simulink model "pmpc_mil_nu"  (R2024b)
settings: Solver=ode1  StartTime=0  StopTime=20  FixedStep=0.001  RelTol=1e-3
PreLoadFcn:
  | root = 'D:\OneDrive - mail.scut.edu.cn\Thesis\Code\Controller\MAIN\experiments\nonuniform_grid_20261115';
  | 
  | addpath(fullfile(root,'pmpc_core'),'-begin');
  | addpath(fullfile(root,'nlcsnn'),'-begin');
values from neighbouring files (symbols this model uses):
  a_pl = exp(-Tc/tau_e)    [init_valve2.m]
  b_pl = (Vdc/R)*(1 - a_pl)    [init_valve2.m]
  Iref_init = 0    [init_valve2.m]
  Ki = wc*R/Vdc    (= 26.1799387799)    [init_valve2.m]
  Kp = Ti_ratio*wc*L_H/Vdc    (= 0.0418879020479)    [init_valve2.m]
  Tc = 1/fs_ctrl    (= 0.001)    [init_valve2.m]
  Ts_avg = Tc    (= 0.001)    [init_valve2.m]
undefined symbols (not defined in the file or in its folder): delta_d, dspblkCoreblockFVToolHelper, gcbh, params, Reftraj, state0, V_target
libraries: slpidlib x5, Solver_SF x1
settings Model: Creator=user  LastModifiedBy=user
settings OptimizationCC: ZeroExternalMemoryAtStartup=off  ZeroInternalMemoryAtStartup=off
settings RTWCC: TargetLang=C++
settings GRTTargetCC: TargetLangStandard=C++11 (ISO)  CodeInterfacePackaging=C++ class

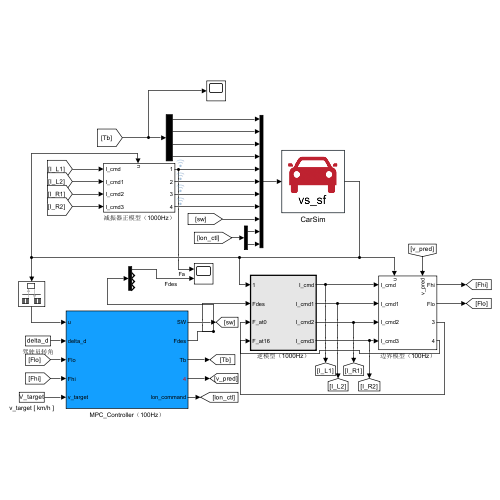
[thumbnail: Simulink's stored preview of the top-level diagram]
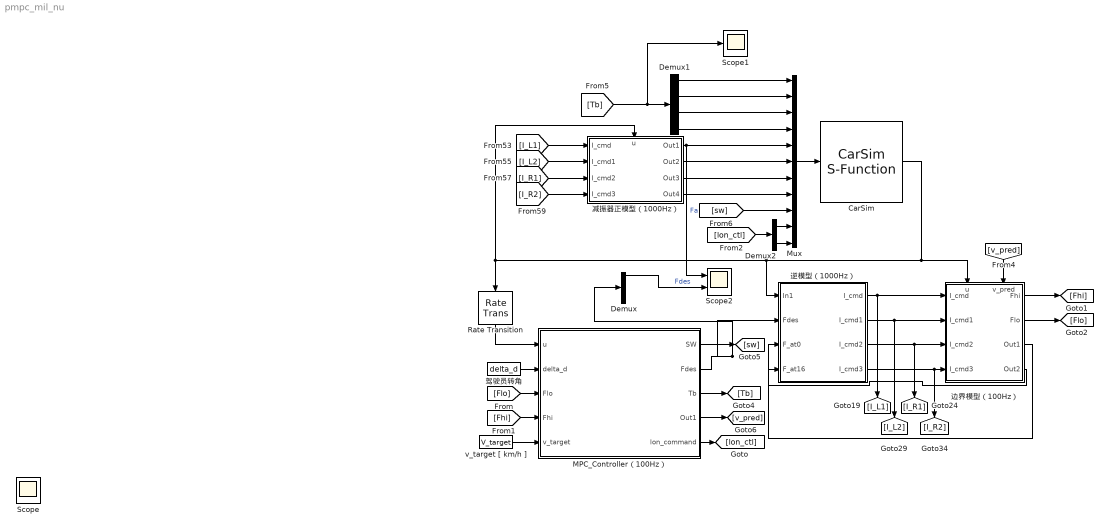
== system pmpc_mil_nu ==
  CarSim : Solver_SF/CarSim S-Function  Priority=1  SIMFILE=simfile.sim
  Demux : Demux
  Demux1 : Demux
  Demux2 : Demux  Outputs=2
  MPC_Controller（100Hz） : Subsystem  SystemSampleTime=0.01
  Mux : Mux  Inputs=11
  Rate Transition : RateTransition  OutPortSampleTime=0.01
  Scope1 : Scope
  Scope2 : Scope  NumInputPorts=2
  v_target [ km/h ] : Constant  Value=V_target
  减振器正模型（1000Hz） : Subsystem
      settings: PortSchema="{\"entries\":[{\"content\":{\"sides\":[{\"content\":{\"connectorIds\":[\"In1\",\"In2\",\"In3\",\"In4\"]},\"type\":\"ConnectorPlacement.EquallySpacedRectSide\",\"uuid\":\"6bdae15d-f673-492b-8508-25b25c52f85c\"},{\"content\":{\"connectorIds\":[\"Out1\",\"Out2\",\"Out3\",\"Out4\"],\"side\":\"RIGHT\"},\"type\":\"ConnectorPlacement.EquallySpacedRectSide\",\"uuid\":\"9d0d46be-4d90-4429-bc90-e3747ae06ca5\"},{\"content\":{\"connectorIds\":[\"In5\"],\"side\":\"TOP\"},\"type\":\"ConnectorPlacement.EquallySpacedRectSide\",\"uuid\":\"d2f3a784-c5ed-41f2-ae04-a2222bae6aeb\"}]},\"type\":\"ConnectorPlacement.EquallySpacedConnector\",\"uuid\":\"c35c18e7-51b3-4d33-8294-a9e611d66578\"}],\"packageUris\":[\"http://schema.mathworks.com/mf0/Connector/R2020b\"],\"version\":\"1.0\"}"
  边界模型（100Hz） : Subsystem
      settings: PortSchema="{\"entries\":[{\"content\":{\"sides\":[{\"content\":{\"connectorIds\":[\"In1\",\"In2\",\"In3\",\"In4\"]},\"type\":\"ConnectorPlacement.EquallySpacedRectSide\",\"uuid\":\"717c1422-5e21-4652-bca5-057ad50c6cdf\"},{\"content\":{\"connectorIds\":[\"Out1\",\"Out2\",\"Out3\",\"Out4\"],\"side\":\"RIGHT\"},\"type\":\"ConnectorPlacement.EquallySpacedRectSide\",\"uuid\":\"4ad5078c-896a-44f2-a1cc-d2c9341f0df9\"},{\"content\":{\"connectorIds\":[\"In5\",\"In6\"],\"side\":\"TOP\"},\"type\":\"ConnectorPlacement.EquallySpacedRectSide\",\"uuid\":\"81dc3538-7b06-42f0-8b15-8c4302fdfcb3\"}]},\"type\":\"ConnectorPlacement.EquallySpacedConnector\",\"uuid\":\"666a4fc5-cde4-42f5-84f2-e20b6be44764\"}],\"packageUris\":[\"http://schema.mathworks.com/mf0/Connector/R2020b\"],\"version\":\"1.0\"}"
  逆模型（1000Hz） : Subsystem  TreatAsAtomicUnit=on  SystemSampleTime=0.001
  驾驶员转角 : Constant  Value=delta_d
  Scope : Scope
  wires:
  Mux/1 -> CarSim/1
  [I_L1] -> 减振器正模型（1000Hz）/1(I_cmd)
  [I_L2] -> 减振器正模型（1000Hz）/2(I_cmd1)
  [I_R1] -> 减振器正模型（1000Hz）/3(I_cmd2)
  [I_R2] -> 减振器正模型（1000Hz）/4(I_cmd3)
  [sw] -> Mux/9
  减振器正模型（1000Hz）/1(Out1) -> Mux/5, Scope2/1  "Fa"
  减振器正模型（1000Hz）/2(Out2) -> Mux/6
  减振器正模型（1000Hz）/3(Out3) -> Mux/7
  减振器正模型（1000Hz）/4(Out4) -> Mux/8
  Demux1/1 -> Mux/1
  Demux1/2 -> Mux/2
  Demux1/3 -> Mux/3
  Demux1/4 -> Mux/4
  CarSim/1 -> 边界模型（100Hz）/5(u), 逆模型（1000Hz）/1(In1), 减振器正模型（1000Hz）/5(u), Rate Transition/1
  [Flo] -> MPC_Controller（100Hz）/3(Flo)
  [Fhi] -> MPC_Controller（100Hz）/4(Fhi)
  MPC_Controller（100Hz）/3(Tb) -> [Tb]
  MPC_Controller（100Hz）/1(SW) -> [sw]
  Rate Transition/1 -> MPC_Controller（100Hz）/1(u)
  逆模型（1000Hz）/1(I_cmd) -> [I_L1], 边界模型（100Hz）/1(I_cmd)
  逆模型（1000Hz）/2(I_cmd1) -> [I_L2], 边界模型（100Hz）/2(I_cmd1)
  逆模型（1000Hz）/3(I_cmd2) -> [I_R1], 边界模型（100Hz）/3(I_cmd2)
  逆模型（1000Hz）/4(I_cmd3) -> [I_R2], 边界模型（100Hz）/4(I_cmd3)
  MPC_Controller（100Hz）/2(Fdes) -> Demux/1, 逆模型（1000Hz）/2(Fdes)
  v_target [ km/h ]/1 -> MPC_Controller（100Hz）/5(v_target)
  [Tb] -> Scope1/1, Demux1/1
  边界模型（100Hz）/1(Fhi) -> [Fhi]
  边界模型（100Hz）/2(Flo) -> [Flo]
  MPC_Controller（100Hz）/4(Out1) -> [v_pred]
  [v_pred] -> 边界模型（100Hz）/6(v_pred)
  Demux/1 -> Scope2/2  "Fdes"
  MPC_Controller（100Hz）/5(lon_command) -> [lon_ctl]
  Demux2/1 -> Mux/10
  Demux2/2 -> Mux/11
  [lon_ctl] -> Demux2/1
  驾驶员转角/1 -> MPC_Controller（100Hz）/2(delta_d)
  边界模型（100Hz）/3(Out1) -> 逆模型（1000Hz）/3(F_at0)
  边界模型（100Hz）/4(Out2) -> 逆模型（1000Hz）/4(F_at16)

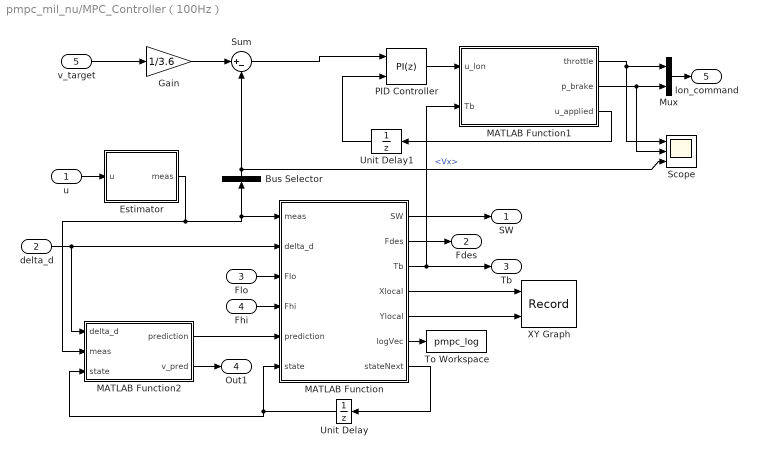
== system pmpc_mil_nu/MPC_Controller（100Hz） ==
  u : Inport
  delta_d : Inport  Port=2
  Flo : Inport  Port=3
  Fhi : Inport  Port=4
  v_target : Inport  Port=5
  Bus Selector : BusSelector  OutputSignals=Vx
  Estimator : MATLAB Function  TreatAsAtomicUnit=on
  Gain : Gain  Gain=1/3.6
  MATLAB Function : MATLAB Function  TreatAsAtomicUnit=on
  MATLAB Function1 : MATLAB Function  TreatAsAtomicUnit=on
  MATLAB Function2 : MATLAB Function  TreatAsAtomicUnit=on
  Mux : Mux  Inputs=2
  PID Controller : slpidlib/PID Controller  Controller=PI  Form=Parallel  TimeDomain=Discrete-time  UseExternalTs=off  SampleTime=-1  IntegratorMethod=Forward Euler  FilterMethod=Forward Euler  ControllerParametersSource=internal  P=0.2  I=0.005  UseKiTs=off  D=0  UseExternalDerivativeSource=off  N=100  UseFilter=on  TunerSelectOption=Transfer Function Based (PID Tuner App)  InitialConditionSource=internal  InitialConditionForIntegrator=0  InitialConditionForFilter=0  DifferentiatorICPrevScaledInput=0  ExternalReset=none  TrackingMode=on  Kt=1  LimitOutput=on  SatLimitsSource=internal  UpperSaturationLimit=1  LowerSaturationLimit=-1  LinearizeAsGain=on  AntiWindupMode=back-calculation  Kb=1  LimitIntegrator=off  UpperIntegratorSaturationLimit=inf  LowerIntegratorSaturationLimit=-inf  POutMin=[]  POutMax=[]  IOutMin=[]  IOutMax=[]  DOutMin=[]  DOutMax=[]  NOutMin=[]  NOutMax=[]  SumOutMin=[]  SumOutMax=[]  SaturationOutMin=[]  SaturationOutMax=[]  PParamMin=[]  PParamMax=[]  IParamMin=[]  IParamMax=[]  DParamMin=[]  DParamMax=[]  NParamMin=[]  NParamMax=[]  KbParamMin=[]  KbParamMax=[]  KtParamMin=[]  KtParamMax=[]  KbOutMin=[]  KbOutMax=[]  KtOutMin=[]  KtOutMax=[]  IntegratorOutMin=[]  IntegratorOutMax=[]  FilterOutMin=[]  FilterOutMax=[]  SumI1OutMin=[]  SumI1OutMax=[]  SumI2OutMin=[]  SumI2OutMax=[]  SumI3OutMin=[]  SumI3OutMax=[]  SumI4OutMin=[]  SumI4OutMax=[]  SumDOutMin=[]  SumDOutMax=[]  DifferentiatorOutMin=[]  DifferentiatorOutMax=[]  FilterDiffOutCoefMin=[]  FilterDiffOutCoefMax=[]  ReciprocalOutMin=[]  ReciprocalOutMax=[]  SumDenOutMin=[]  SumDenOutMax=[]  SumNumOutMin=[]  SumNumOutMax=[]  DivideOutMin=[]  DivideOutMax=[]  UdiffTsProdOutMin=[]  UdiffTsProdOutMax=[]  NTsProdOutMin=[]  NTsProdOutMax=[]  UintegralTsProdOutMin=[]  UintegralTsProdOutMax=[]  UngainTsProdOutMin=[]  UngainTsProdOutMax=[]  ClampingZeroOutDataTypeStr=Inherit: Inherit via back propagation  ClampingZeroOutMin=[]  ClampingZeroOutMax=[]  FilterDenConstantOutDataTypeStr=Inherit: Inherit via back propagation  FilterDenConstantOutMin=[]  FilterDenConstantOutMax=[]  PCopyOutDataTypeStr=Inherit: Inherit via back propagation  PCopyOutMin=[]  PCopyOutMax=[]  NCopyOutDataTypeStr=Inherit: Inherit via back propagation  NCopyOutMin=[]  NCopyOutMax=[]  IntegratorContinuousStateAttributes=''  IntegratorStateMustResolveToSignalObject=off  IntegratorRTWStateStorageClass=Auto  FilterContinuousStateAttributes=''  FilterStateMustResolveToSignalObject=off  FilterRTWStateStorageClass=Auto  ParallelPVariant=InternalParameters  IdealPVariant=Disabled  IVariant=InternalParameters  DVariant=Disabled  IntegratorVariant=Discrete  SatVariant=Enabled  AWVariant=BackCalculation  PCopyVariant=Disabled  TRVariant=Enabled  FdbkBlocksVariant=Forward  IdealPFdbkVariant=Disabled  SatFdbkVariant=Disabled  DerivativeFilterVariant=Disabled  NVariant=Disabled  NCopyVariant=Disabled_SignalSpec  FilterICVariant=Disabled  IntegratorICVariant=InternalICs  ExternalResetVariant=Disabled  TRSumVariant=TrackingMode  SumFdbkVariant=Disabled  SumVariant=Sum_PI  TsampFilterVariant=InternalTs  TsampNgainVariant=Passthrough  TsampIntegralVariant=Disabled_SignalSpec  ExternalSaturationOutDataTypeStr=Inherit: Same as second input  DerivativeSourceVariant=Disabled  PreIntVariant=InternalPreInt
  Scope : Scope  NumInputPorts=3
  Sum : Sum  Inputs=|+-
  To Workspace : ToWorkspace  VariableName=pmpc_log  SaveFormat=Timeseries  SampleTime=-1
  Unit Delay : UnitDelay  InitialCondition=state0  SampleTime=0.01  HasFrameUpgradeWarning=on
  Unit Delay1 : UnitDelay  SampleTime=-1  HasFrameUpgradeWarning=on
  XY Graph : Record  FileSettingsInternal="{\"entries\":[{\"content\":{\"excelSettings\":{\"content\":{},\"type\":\"Streamout.ExcelSettings\"}},\"type\":\"Streamout.FileSettingStorage\",\"uuid\":\"\"}],\"packageUris\":[\"http:\\/\\/schema.mathworks.com\\/mf0\\/streamout_blocks\\/R2020a\"],\"version\":\"1.0\"}"  Layout=[1 1]  SignalsInternal="{\"entries\":[{\"content\":{\"signals\":[{\"content\":{\"blockPath\":[],\"dimensions\":[1],\"domain\":\"\",\"lineColor\":\"#a2142f\",\"lineWidth\":2,\"plots\":[ 1 ],\"port\":1,\"signalID\":1,\"signalName\":\"MATLAB Function:4\"},\"type\":\"RecordBlkView.Signal\",\"uuid\":\"\"},{\"content\":{\"blockPath\":[],\"dimensions\":[1],\"domain\":\"\",\"lineColor\":\"#139fff\",\"lineWidth\":2,\"plots\":[ 1 ],\"port\":2,\"signalID\":2,\"signalName\":\"MATLAB Function:5\"},\"type\":\"RecordBlkView.Signal\",\"uuid\":\"\"}]},\"type\":\"RecordBlkView.InputSignals\",\"uuid\":\"\"}],\"packageUris\":[\"http:\\/\\/schema.mathworks.com\\/mf0\\/streamout_blocks\\/R2020a\"],\"version\":\"1.0\"}"  VisualizationBindings="{\"xyplotplugin\":{\"info\":[{\"series\":[{\"bindingParametersList\":[{\"parameter\":\"X-Axis\",\"signalID\":1,\"signalName\":\"MATLAB Function:4\"},{\"parameter\":\"Y-Axis\",\"signalID\":2,\"signalName\":\"MATLAB Function:5\"}],\"seriesID\":0}],\"subplotID\":1}]}}"  CompatibilityTag=XY
  SW : Outport
  Fdes : Outport  Port=2
  Tb : Outport  Port=3
  Out1 : Outport  Port=4
  lon_command : Outport  Port=5
  wires:
  u/1 -> Estimator/1(u)
  Estimator/1(meas) -> MATLAB Function2/2(meas), Bus Selector/1, MATLAB Function/1(meas)
  Unit Delay/1 -> MATLAB Function/6(state), MATLAB Function2/3(state)
  MATLAB Function/7(stateNext) -> Unit Delay/1
  Flo/1 -> MATLAB Function/3(Flo)
  Fhi/1 -> MATLAB Function/4(Fhi)
  Sum/1 -> PID Controller/1
  PID Controller/1 -> MATLAB Function1/1(u_lon)
  Bus Selector/1 -> Sum/2, Scope/3  "<Vx>"
  v_target/1 -> Gain/1
  MATLAB Function1/2(p_brake) -> Mux/2, Scope/2
  Gain/1 -> Sum/1
  MATLAB Function1/3(u_applied) -> Unit Delay1/1
  Unit Delay1/1 -> PID Controller/2
  MATLAB Function1/1(throttle) -> Mux/1, Scope/1
  MATLAB Function/1(SW) -> SW/1
  MATLAB Function/3(Tb) -> Tb/1, MATLAB Function1/2(Tb)
  MATLAB Function/2(Fdes) -> Fdes/1
  MATLAB Function/4(Xlocal) -> XY Graph/1
  MATLAB Function/5(Ylocal) -> XY Graph/2
  MATLAB Function2/1(prediction) -> MATLAB Function/5(prediction)
  MATLAB Function2/2(v_pred) -> Out1/1
  Mux/1 -> lon_command/1
  MATLAB Function/6(logVec) -> To Workspace/1
  delta_d/1 -> MATLAB Function2/1(delta_d), MATLAB Function/2(delta_d)

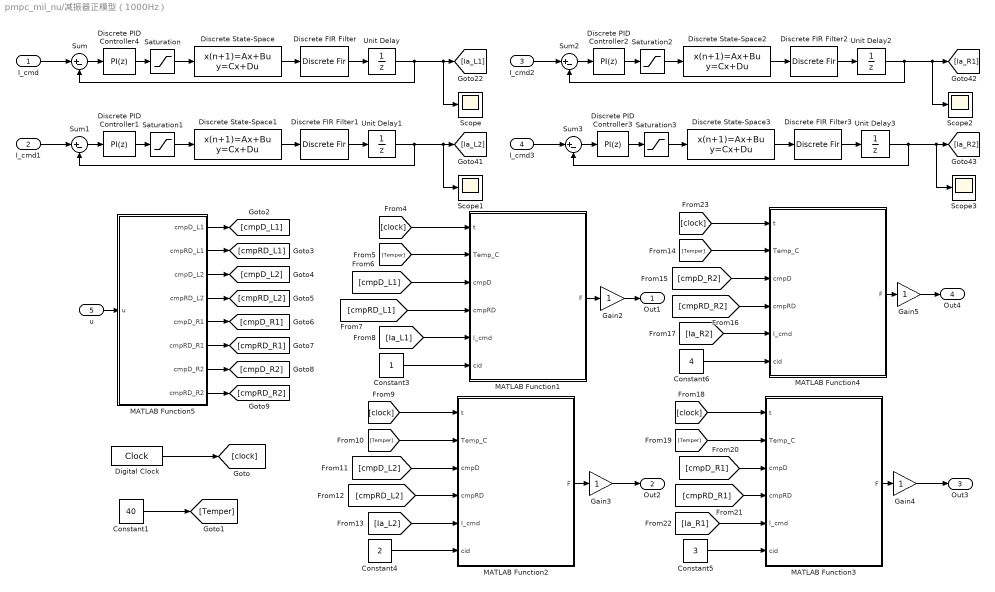
== system pmpc_mil_nu/减振器正模型（1000Hz） ==
  I_cmd : Inport
  I_cmd1 : Inport  Port=2
  I_cmd2 : Inport  Port=3
  I_cmd3 : Inport  Port=4
  u : Inport  Port=5
  Constant1 : Constant  Value=40
  Constant3 : Constant
  Constant4 : Constant  Value=2
  Constant5 : Constant  Value=3
  Constant6 : Constant  Value=4
  Digital Clock : DigitalClock  SampleTime=0.001
  Discrete FIR Filter{,1..3} (4 alike) : DiscreteFir  LoadFcn=dspblkCoreblockFVToolHelper(gcbh,'load');  InitialStates=Iref_init
      settings: CopyFcn=dspblkCoreblockFVToolHelper(gcbh,'copy');  DeleteFcn=dspblkCoreblockFVToolHelper(gcbh,'close');  ModelCloseFcn=dspblkCoreblockFVToolHelper(gcbh,'close');  PreSaveFcn=dspblkCoreblockFVToolHelper(gcbh,'presave');  PostSaveFcn=dspblkCoreblockFVToolHelper(gcbh,'postsave');  CloseFcn=dspblkCoreblockFVToolHelper(gcbh,'close');
  Discrete PID Controller{1..4} (4 alike) : slpidlib/PID Controller  Controller=PI  Form=Parallel  TimeDomain=Discrete-time  UseExternalTs=off  SampleTime=Tc  IntegratorMethod=Forward Euler  FilterMethod=Forward Euler  ControllerParametersSource=internal  P=Kp  I=Ki  UseKiTs=off  D=0  UseExternalDerivativeSource=off  N=100  UseFilter=on  TunerSelectOption=Transfer Function Based (PID Tuner App)  InitialConditionSource=internal  InitialConditionForIntegrator=D_init  InitialConditionForFilter=0  DifferentiatorICPrevScaledInput=0  ExternalReset=none  TrackingMode=off  Kt=1  LimitOutput=on  SatLimitsSource=internal  UpperSaturationLimit=1  LowerSaturationLimit=0  LinearizeAsGain=off  AntiWindupMode=clamping  Kb=1  LimitIntegrator=off  UpperIntegratorSaturationLimit=duty_max − u_ff  LowerIntegratorSaturationLimit=duty_min − u_ff  POutMin=[]  POutMax=[]  IOutMin=[]  IOutMax=[]  DOutMin=[]  DOutMax=[]  NOutMin=[]  NOutMax=[]  SumOutMin=[]  SumOutMax=[]  SaturationOutMin=[]  SaturationOutMax=[]  PParamMin=[]  PParamMax=[]  IParamMin=[]  IParamMax=[]  DParamMin=[]  DParamMax=[]  NParamMin=[]  NParamMax=[]  KbParamMin=[]  KbParamMax=[]  KtParamMin=[]  KtParamMax=[]  KbOutMin=[]  KbOutMax=[]  KtOutMin=[]  KtOutMax=[]  IntegratorOutMin=[]  IntegratorOutMax=[]  FilterOutMin=[]  FilterOutMax=[]  SumI1OutMin=[]  SumI1OutMax=[]  SumI2OutMin=[]  SumI2OutMax=[]  SumI3OutMin=[]  SumI3OutMax=[]  SumI4OutMin=[]  SumI4OutMax=[]  SumDOutMin=[]  SumDOutMax=[]  DifferentiatorOutMin=[]  DifferentiatorOutMax=[]  FilterDiffOutCoefMin=[]  FilterDiffOutCoefMax=[]  ReciprocalOutMin=[]  ReciprocalOutMax=[]  SumDenOutMin=[]  SumDenOutMax=[]  SumNumOutMin=[]  SumNumOutMax=[]  DivideOutMin=[]  DivideOutMax=[]  UdiffTsProdOutMin=[]  UdiffTsProdOutMax=[]  NTsProdOutMin=[]  NTsProdOutMax=[]  UintegralTsProdOutMin=[]  UintegralTsProdOutMax=[]  UngainTsProdOutMin=[]  UngainTsProdOutMax=[]  ClampingZeroOutDataTypeStr=Inherit: Inherit via back propagation  ClampingZeroOutMin=[]  ClampingZeroOutMax=[]  FilterDenConstantOutDataTypeStr=Inherit: Inherit via back propagation  FilterDenConstantOutMin=[]  FilterDenConstantOutMax=[]  PCopyOutDataTypeStr=Inherit: Inherit via back propagation  PCopyOutMin=[]  PCopyOutMax=[]  NCopyOutDataTypeStr=Inherit: Inherit via back propagation  NCopyOutMin=[]  NCopyOutMax=[]  IntegratorContinuousStateAttributes=''  IntegratorStateMustResolveToSignalObject=off  IntegratorRTWStateStorageClass=Auto  FilterContinuousStateAttributes=''  FilterStateMustResolveToSignalObject=off  FilterRTWStateStorageClass=Auto  ParallelPVariant=InternalParameters  IdealPVariant=Disabled  IVariant=InternalParameters  DVariant=Disabled  IntegratorVariant=Discrete  SatVariant=Enabled  AWVariant=DiscClampingParallel  PCopyVariant=Disabled  TRVariant=Disabled  FdbkBlocksVariant=Forward  IdealPFdbkVariant=Disabled  SatFdbkVariant=Disabled  DerivativeFilterVariant=Disabled  NVariant=Disabled  NCopyVariant=Disabled_SignalSpec  FilterICVariant=Disabled  IntegratorICVariant=InternalICs  ExternalResetVariant=Disabled  TRSumVariant=Passthrough  SumFdbkVariant=Disabled  SumVariant=Sum_PI  TsampFilterVariant=InternalTs  TsampNgainVariant=Passthrough  TsampIntegralVariant=Disabled_SignalSpec  ExternalSaturationOutDataTypeStr=Inherit: Same as second input  DerivativeSourceVariant=Disabled  PreIntVariant=InternalPreInt
      settings: LibrarySourceBlock=simulink/Discrete/Discrete PID Controller
  Discrete State-Space{,1..3} (4 alike) : DiscreteStateSpace  A=a_pl  B=b_pl  D=0  InitialCondition=Iref_init  SampleTime=Ts_avg
  Gain{2..5} (4 alike) : Gain
  MATLAB Function1 : MATLAB Function  TreatAsAtomicUnit=on
  MATLAB Function2 : MATLAB Function  TreatAsAtomicUnit=on
  MATLAB Function3 : MATLAB Function  TreatAsAtomicUnit=on
  MATLAB Function4 : MATLAB Function  TreatAsAtomicUnit=on
  MATLAB Function5 : MATLAB Function  TreatAsAtomicUnit=on
  Saturation{,1..3} (4 alike) : Saturate  UpperLimit=1  LowerLimit=0
  Scope{,1..3} (4 alike) : Scope
  Sum{,1..3} (4 alike) : Sum  Inputs=|+-
  Unit Delay{,1..3} (4 alike) : UnitDelay  InitialCondition=Iref_init  SampleTime=1e-3  HasFrameUpgradeWarning=on
  Out1 : Outport
  Out2 : Outport  Port=2
  Out3 : Outport  Port=3
  Out4 : Outport  Port=4
  wires:
  [clock] -> MATLAB Function4/1(t)
  [Ia_R2] -> MATLAB Function4/5(I_cmd)
  Constant5/1 -> MATLAB Function3/6(cid)
  [Temper] -> MATLAB Function1/2(Temp_C)
  MATLAB Function1/1(F) -> Gain2/1
  [cmpRD_R1] -> MATLAB Function3/4(cmpRD)
  [Ia_R1] -> MATLAB Function3/5(I_cmd)
  [Ia_L1] -> MATLAB Function1/5(I_cmd)
  [clock] -> MATLAB Function3/1(t)
  [Ia_L2] -> MATLAB Function2/5(I_cmd)
  Constant4/1 -> MATLAB Function2/6(cid)
  MATLAB Function2/1(F) -> Gain3/1
  [cmpD_R2] -> MATLAB Function4/3(cmpD)
  Digital Clock/1 -> [clock]
  Gain3/1 -> Out2/1
  [cmpRD_L1] -> MATLAB Function1/4(cmpRD)
  Gain5/1 -> Out4/1
  [Temper] -> MATLAB Function3/2(Temp_C)
  MATLAB Function3/1(F) -> Gain4/1
  Constant1/1 -> [Temper]
  [cmpRD_L2] -> MATLAB Function2/4(cmpRD)
  [cmpD_R1] -> MATLAB Function3/3(cmpD)
  [cmpRD_R2] -> MATLAB Function4/4(cmpRD)
  Gain4/1 -> Out3/1
  [clock] -> MATLAB Function1/1(t)
  MATLAB Function4/1(F) -> Gain5/1
  [cmpD_L1] -> MATLAB Function1/3(cmpD)
  Gain2/1 -> Out1/1
  Constant6/1 -> MATLAB Function4/6(cid)
  [Temper] -> MATLAB Function2/2(Temp_C)
  Constant3/1 -> MATLAB Function1/6(cid)
  [Temper] -> MATLAB Function4/2(Temp_C)
  [clock] -> MATLAB Function2/1(t)
  [cmpD_L2] -> MATLAB Function2/3(cmpD)
  u/1 -> MATLAB Function5/1(u)
  MATLAB Function5/1(cmpD_L1) -> [cmpD_L1]
  MATLAB Function5/2(cmpRD_L1) -> [cmpRD_L1]
  MATLAB Function5/3(cmpD_L2) -> [cmpD_L2]
  MATLAB Function5/4(cmpRD_L2) -> [cmpRD_L2]
  MATLAB Function5/5(cmpD_R1) -> [cmpD_R1]
  MATLAB Function5/6(cmpRD_R1) -> [cmpRD_R1]
  MATLAB Function5/7(cmpD_R2) -> [cmpD_R2]
  MATLAB Function5/8(cmpRD_R2) -> [cmpRD_R2]
  I_cmd/1 -> Sum/1
  Sum/1 -> Discrete PID Controller4/1
  Unit Delay/1 -> Scope/1, [Ia_L1], Sum/2
  Discrete FIR Filter/1 -> Unit Delay/1
  Discrete PID Controller4/1 -> Saturation/1
  Discrete State-Space/1 -> Discrete FIR Filter/1
  Saturation/1 -> Discrete State-Space/1
  Unit Delay1/1 -> [Ia_L2], Scope1/1, Sum1/2
  Discrete State-Space1/1 -> Discrete FIR Filter1/1
  Discrete FIR Filter1/1 -> Unit Delay1/1
  Saturation1/1 -> Discrete State-Space1/1
  Sum1/1 -> Discrete PID Controller1/1
  Discrete PID Controller1/1 -> Saturation1/1
  Unit Delay2/1 -> [Ia_R1], Scope2/1, Sum2/2
  Discrete State-Space2/1 -> Discrete FIR Filter2/1
  Discrete FIR Filter2/1 -> Unit Delay2/1
  Saturation2/1 -> Discrete State-Space2/1
  Sum2/1 -> Discrete PID Controller2/1
  Discrete PID Controller2/1 -> Saturation2/1
  Unit Delay3/1 -> [Ia_R2], Scope3/1, Sum3/2
  Discrete State-Space3/1 -> Discrete FIR Filter3/1
  Discrete FIR Filter3/1 -> Unit Delay3/1
  Saturation3/1 -> Discrete State-Space3/1
  Sum3/1 -> Discrete PID Controller3/1
  I_cmd3/1 -> Sum3/1
  Discrete PID Controller3/1 -> Saturation3/1
  I_cmd1/1 -> Sum1/1
  I_cmd2/1 -> Sum2/1

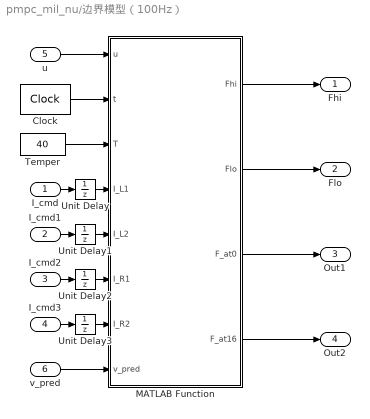
== system pmpc_mil_nu/边界模型（100Hz） ==
  I_cmd : Inport
  I_cmd1 : Inport  Port=2
  I_cmd2 : Inport  Port=3
  I_cmd3 : Inport  Port=4
  u : Inport  Port=5
  v_pred : Inport  Port=6
  Clock : DigitalClock  SampleTime=0.001
  MATLAB Function : MATLAB Function  TreatAsAtomicUnit=on
  Temper : Constant  Value=40
  Unit Delay{,1..3} (4 alike) : UnitDelay  SampleTime=0.001  HasFrameUpgradeWarning=on
  Fhi : Outport
  Flo : Outport  Port=2
  Out1 : Outport  Port=3
  Out2 : Outport  Port=4
  wires:
  Temper/1 -> MATLAB Function/3(T)
  Clock/1 -> MATLAB Function/2(t)
  v_pred/1 -> MATLAB Function/8(v_pred)
  u/1 -> MATLAB Function/1(u)
  MATLAB Function/1(Fhi) -> Fhi/1
  MATLAB Function/2(Flo) -> Flo/1
  I_cmd/1 -> Unit Delay/1
  Unit Delay/1 -> MATLAB Function/4(I_L1)
  I_cmd1/1 -> Unit Delay1/1
  Unit Delay1/1 -> MATLAB Function/5(I_L2)
  I_cmd2/1 -> Unit Delay2/1
  Unit Delay2/1 -> MATLAB Function/6(I_R1)
  I_cmd3/1 -> Unit Delay3/1
  Unit Delay3/1 -> MATLAB Function/7(I_R2)
  MATLAB Function/3(F_at0) -> Out1/1
  MATLAB Function/4(F_at16) -> Out2/1

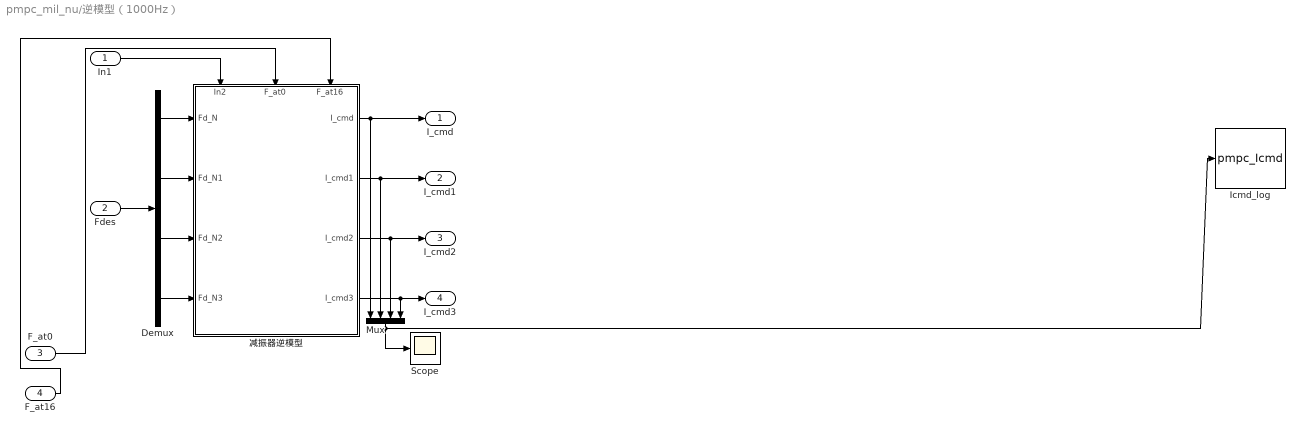
== system pmpc_mil_nu/逆模型（1000Hz） ==
  In1 : Inport
  Fdes : Inport  Port=2
  F_at0 : Inport  Port=3
  F_at16 : Inport  Port=4
  Demux : Demux
  Icmd_log : ToWorkspace  VariableName=pmpc_Icmd  SaveFormat=Structure With Time  SampleTime=-1
  Mux : Mux
  Scope : Scope
  减振器逆模型 : Subsystem
      settings: PortSchema="{\"entries\":[{\"content\":{\"sides\":[{\"content\":{\"connectorIds\":[\"In1\",\"In2\",\"In3\",\"In4\"]},\"type\":\"ConnectorPlacement.EquallySpacedRectSide\",\"uuid\":\"1b1e3cbb-ab52-4b5e-a8c1-091191c7a0a1\"},{\"content\":{\"connectorIds\":[\"Out1\",\"Out2\",\"Out3\",\"Out4\"],\"side\":\"RIGHT\"},\"type\":\"ConnectorPlacement.EquallySpacedRectSide\",\"uuid\":\"e36391e6-cb8e-45c5-b600-19fb73252ab2\"},{\"content\":{\"connectorIds\":[\"In5\",\"In6\",\"In7\"],\"side\":\"TOP\"},\"type\":\"ConnectorPlacement.EquallySpacedRectSide\",\"uuid\":\"92f6e0c3-7b8a-4a08-9013-fccb1e083f6f\"}]},\"type\":\"ConnectorPlacement.EquallySpacedConnector\",\"uuid\":\"3214107d-4344-4e68-82b7-79bb17f5024d\"}],\"packageUris\":[\"http://schema.mathworks.com/mf0/Connector/R2020b\"],\"version\":\"1.0\"}"
  I_cmd : Outport
  I_cmd1 : Outport  Port=2
  I_cmd2 : Outport  Port=3
  I_cmd3 : Outport  Port=4
  wires:
  Demux/2 -> 减振器逆模型/2(Fd_N1)
  Demux/4 -> 减振器逆模型/4(Fd_N3)
  减振器逆模型/2(I_cmd1) -> I_cmd1/1, Mux/2
  Demux/1 -> 减振器逆模型/1(Fd_N)
  Demux/3 -> 减振器逆模型/3(Fd_N2)
  In1/1 -> 减振器逆模型/5(In2)
  减振器逆模型/1(I_cmd) -> I_cmd/1, Mux/1
  减振器逆模型/4(I_cmd3) -> I_cmd3/1, Mux/4
  减振器逆模型/3(I_cmd2) -> I_cmd2/1, Mux/3
  Fdes/1 -> Demux/1
  Mux/1 -> Scope/1, Icmd_log/1
  F_at0/1 -> 减振器逆模型/6(F_at0)
  F_at16/1 -> 减振器逆模型/7(F_at16)

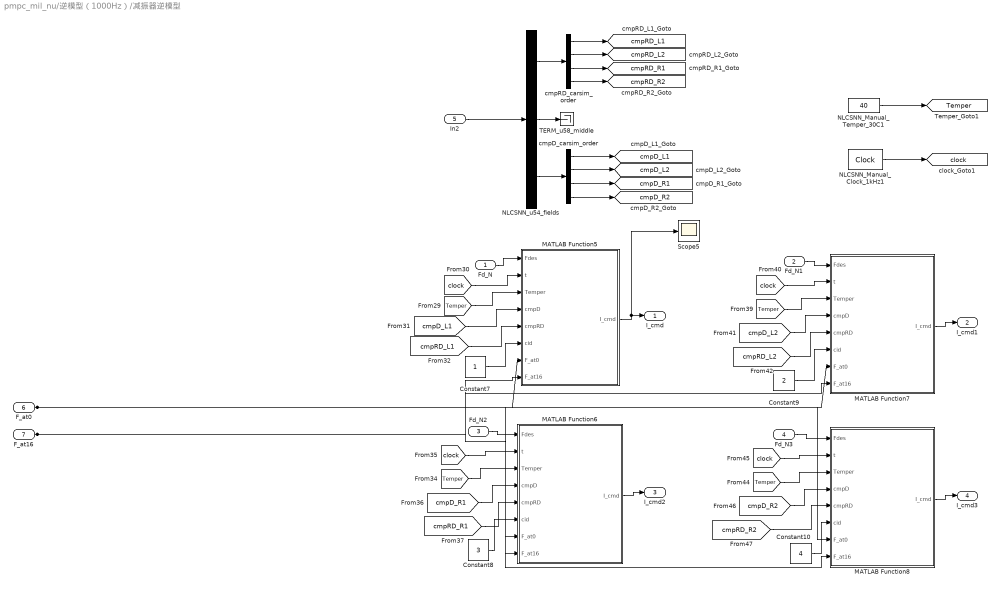
== system pmpc_mil_nu/逆模型（1000Hz）/减振器逆模型 ==
  Fd_N : Inport
  Fd_N1 : Inport  Port=2
  Fd_N2 : Inport  Port=3
  Fd_N3 : Inport  Port=4
  In2 : Inport  Port=5
  F_at0 : Inport  Port=6
  F_at16 : Inport  Port=7
  Constant10 : Constant  Value=4
  Constant7 : Constant
  Constant8 : Constant  Value=3
  Constant9 : Constant  Value=2
  MATLAB Function5 : MATLAB Function  TreatAsAtomicUnit=on
  MATLAB Function6 : MATLAB Function  TreatAsAtomicUnit=on
  MATLAB Function7 : MATLAB Function  TreatAsAtomicUnit=on
  MATLAB Function8 : MATLAB Function  TreatAsAtomicUnit=on
  NLCSNN_Manual_Clock_1kHz1 : DigitalClock  SampleTime=0.001
  NLCSNN_Manual_Temper_30C1 : Constant  Value=40
  NLCSNN_u54_fields : Demux  Outputs=[4 46 4]
  Scope5 : Scope
  TERM_u58_middle : Terminator
  cmpD_carsim_order : Demux
  cmpRD_carsim_order : Demux
  I_cmd : Outport
  I_cmd1 : Outport  Port=2
  I_cmd2 : Outport  Port=3
  I_cmd3 : Outport  Port=4
  tag scope: Temper=global, clock=global, cmpD_L1=global, cmpD_L2=global, cmpD_R1=global, cmpD_R2=global, cmpRD_L1=global, cmpRD_L2=global, cmpRD_R1=global, cmpRD_R2=global
  wires:
  [cmpD_R2] -> MATLAB Function8/4(cmpD)
  [Temper] -> MATLAB Function6/3(Temper)
  In2/1 -> NLCSNN_u54_fields/1
  Constant9/1 -> MATLAB Function7/6(cid)
  [cmpRD_R1] -> MATLAB Function6/5(cmpRD)
  [Temper] -> MATLAB Function5/3(Temper)
  [clock] -> MATLAB Function8/2(t)
  NLCSNN_u54_fields/1 -> cmpRD_carsim_order/1
  Fd_N/1 -> MATLAB Function5/1(Fdes)
  [cmpD_L1] -> MATLAB Function5/4(cmpD)
  cmpD_carsim_order/2 -> [cmpD_L2]
  NLCSNN_u54_fields/2 -> TERM_u58_middle/1
  Fd_N2/1 -> MATLAB Function6/1(Fdes)
  Constant8/1 -> MATLAB Function6/6(cid)
  [cmpRD_L1] -> MATLAB Function5/5(cmpRD)
  cmpRD_carsim_order/4 -> [cmpRD_R2]
  cmpRD_carsim_order/2 -> [cmpRD_L2]
  cmpD_carsim_order/1 -> [cmpD_L1]
  MATLAB Function7/1(I_cmd) -> I_cmd1/1
  MATLAB Function5/1(I_cmd) -> I_cmd/1, Scope5/1
  cmpRD_carsim_order/1 -> [cmpRD_L1]
  cmpD_carsim_order/3 -> [cmpD_R1]
  cmpRD_carsim_order/3 -> [cmpRD_R1]
  NLCSNN_u54_fields/3 -> cmpD_carsim_order/1
  cmpD_carsim_order/4 -> [cmpD_R2]
  [clock] -> MATLAB Function5/2(t)
  [clock] -> MATLAB Function6/2(t)
  [cmpRD_L2] -> MATLAB Function7/5(cmpRD)
  [clock] -> MATLAB Function7/2(t)
  Constant7/1 -> MATLAB Function5/6(cid)
  [cmpRD_R2] -> MATLAB Function8/5(cmpRD)
  Constant10/1 -> MATLAB Function8/6(cid)
  [Temper] -> MATLAB Function7/3(Temper)
  NLCSNN_Manual_Clock_1kHz1/1 -> [clock]
  NLCSNN_Manual_Temper_30C1/1 -> [Temper]
  [Temper] -> MATLAB Function8/3(Temper)
  [cmpD_R1] -> MATLAB Function6/4(cmpD)
  [cmpD_L2] -> MATLAB Function7/4(cmpD)
  MATLAB Function8/1(I_cmd) -> I_cmd3/1
  Fd_N1/1 -> MATLAB Function7/1(Fdes)
  Fd_N3/1 -> MATLAB Function8/1(Fdes)
  MATLAB Function6/1(I_cmd) -> I_cmd2/1
  F_at0/1 -> MATLAB Function5/7(F_at0), MATLAB Function6/7(F_at0), MATLAB Function7/7(F_at0), MATLAB Function8/7(F_at0)
  F_at16/1 -> MATLAB Function5/8(F_at16), MATLAB Function6/8(F_at16), MATLAB Function7/8(F_at16), MATLAB Function8/8(F_at16)

== matlab function pmpc_mil_nu/逆模型（1000Hz）/减振器逆模型/MATLAB Function5 ==
  data: Fdes input; I_cmd output; t input; Temper input; cmpD input; cmpRD input; cid input; F_at0 input; F_at16 input
function I_cmd = fcn(Fdes,t,Temper,cmpD,cmpRD,cid,F_at0,F_at16)
%#codegen
I_cmd = inv_current_impl_10ms(Fdes,t,Temper,cmpD,cmpRD,cid,F_at0(cid),F_at16(cid));
end

== matlab function pmpc_mil_nu/逆模型（1000Hz）/减振器逆模型/MATLAB Function6 ==
  data: Fdes input; I_cmd output; t input; Temper input; cmpD input; cmpRD input; cid input; F_at0 input; F_at16 input
function I_cmd = fcn(Fdes,t,Temper,cmpD,cmpRD,cid,F_at0,F_at16)
%#codegen
I_cmd = inv_current_impl_10ms(Fdes,t,Temper,cmpD,cmpRD,cid,F_at0(cid),F_at16(cid));
end

== matlab function pmpc_mil_nu/逆模型（1000Hz）/减振器逆模型/MATLAB Function7 ==
  data: Fdes input; I_cmd output; t input; Temper input; cmpD input; cmpRD input; cid input; F_at0 input; F_at16 input
function I_cmd = fcn(Fdes,t,Temper,cmpD,cmpRD,cid,F_at0,F_at16)
%#codegen
I_cmd = inv_current_impl_10ms(Fdes,t,Temper,cmpD,cmpRD,cid,F_at0(cid),F_at16(cid));
end

== matlab function pmpc_mil_nu/逆模型（1000Hz）/减振器逆模型/MATLAB Function8 ==
  data: Fdes input; I_cmd output; t input; Temper input; cmpD input; cmpRD input; cid input; F_at0 input; F_at16 input
function I_cmd = fcn(Fdes,t,Temper,cmpD,cmpRD,cid,F_at0,F_at16)
%#codegen
I_cmd = inv_current_impl_10ms(Fdes,t,Temper,cmpD,cmpRD,cid,F_at0(cid),F_at16(cid));
end

== matlab function pmpc_mil_nu/减振器正模型（1000Hz）/MATLAB Function5 ==
  data: u input; cmpD_L1 output; cmpRD_L1 output; cmpD_L2 output; cmpRD_L2 output; cmpD_R1 output; cmpRD_R1 output; cmpD_R2 output; cmpRD_R2 output
function [cmpD_L1,cmpRD_L1,cmpD_L2,cmpRD_L2, ...
          cmpD_R1,cmpRD_R1,cmpD_R2,cmpRD_R2] = fcn(u)
%#codegen
% u：当前 CarSim 54 路输出
% 位移 mm，速度 mm/s，保持原单位

cmpD_L1  = u(51);
cmpRD_L1 = u(1);

cmpD_L2  = u(52);
cmpRD_L2 = u(2);

cmpD_R1  = u(53);
cmpRD_R1 = u(3);

cmpD_R2  = u(54);
cmpRD_R2 = u(4);
end

== matlab function pmpc_mil_nu/MPC_Controller（100Hz）/MATLAB Function1 ==
  data: u_lon input; throttle output; Tb input; p_brake output; u_applied output
function [throttle,p_brake,u_applied] = fcn(u_lon,Tb)
[throttle,p_brake,u_applied] = lon_arbitrate(u_lon,Tb);
end

== matlab function pmpc_mil_nu/MPC_Controller（100Hz）/MATLAB Function2 ==
  settings: updateMethod=DISCRETE  sampleTime=0.01
  data: delta_d input; prediction output Bus: PMPC_PredictionBus; meas input Bus: PMPC_MeasBus; v_pred output; state input Bus: PMPC_StateBus; Reftraj parameter; params parameter
function [prediction,v_pred] = fcn(delta_d, meas,state,Reftraj, params)
%#codegen
[v_pred,prediction] = pmpc_preview(meas,Reftraj,params,state,delta_d);
end

== matlab function pmpc_mil_nu/边界模型（100Hz）/MATLAB Function ==
  data: u input; Fhi output; t input; T input; I_L1 input; I_L2 input; I_R1 input; I_R2 input; v_pred input; Flo output; F_at0 output; F_at16 output; params parameter
function [Fhi,Flo,F_at0,F_at16] = ...
    fcn(u,t,T,I_L1,I_L2,I_R1,I_R2,v_pred, params)
%#codegen
[Fhi,Flo,F_at0,F_at16] = force_bounds_four( ...
    u,t,T,I_L1,I_L2,I_R1,I_R2,v_pred,params);
end

== matlab function pmpc_mil_nu/MPC_Controller（100Hz）/Estimator ==
  data: u input; meas output Bus: PMPC_MeasBus
function meas = fcn(u) %#codegen
%PMPC_MEASURE 当前 CarSim 54 路输出转为 pmpc_step 的 SI 测量结构。
% 输入与 meas 四角向量均为 [L1;L2;R1;R2]。
% 不估计车辆参数
% 固定为列向量，使四角字段为 4x1；deg 转 rad，km/h 转 m/s。
% Fx/Fy/Fz/Fd 单位 N，Td 单位 Nm；delta_front 为左前/右前。
u = double(u(:)); % CarSim 测量和控制器统一使用 double。%转为列向量
meas = struct('X',u(40),'Y',u(41),'Vx',u(42)/3.6,'Vy',u(43)/3.6, ...
    'yaw',u(39)*pi/180,'r',u(34)*pi/180, ...
    'phi',u(38)*pi/180,'p',u(33)*pi/180, ...
    'delta_front',[u(46);u(47)]*pi/180,'steering_wheel',u(48)*pi/180, ...
    'Fx',u(9:12), ...
    'Fy',u(13:16), ...
    'Fz',u(17:20), ...
    'Fd',u(21:24), ...
    'Td',u(29:32), ...
    'vd',u(1:4)/1000); % CMPRD，压缩为正；mm/s -> m/s
end

== matlab function pmpc_mil_nu/MPC_Controller（100Hz）/MATLAB Function ==
  settings: updateMethod=DISCRETE  sampleTime=0.01
  data: SW output double; Fdes output double; meas input Bus: PMPC_MeasBus; delta_d input; Tb output double; Xlocal output; Ylocal output; logVec output size=[27 1]; Flo input; Fhi input; prediction input Bus: PMPC_PredictionBus; state input Bus: PMPC_StateBus; stateNext output Bus: PMPC_StateBus; Reftraj parameter; params parameter
function [SW,Fdes,Tb,Xlocal,Ylocal,logVec,stateNext] = ...
    fcn(meas,delta_d, Flo,Fhi,prediction,state, Reftraj, params)
%#codegen
[SW,Fdes,Tb,stateNext,Xlocal,Ylocal,logVec] =...
    pmpc_step(meas,Reftraj,params,Flo,Fhi,state,prediction,delta_d);
end

== matlab function pmpc_mil_nu/减振器正模型（1000Hz）/MATLAB Function1 ==
  data: t input; F output; Temp_C input; cmpD input; cmpRD input; I_cmd input; cid input
function F = fwd_mf(t, Temp_C, cmpD, cmpRD, I_cmd, cid)
%#codegen
F = fwd_mf_impl(t, Temp_C, cmpD, cmpRD, I_cmd, cid);

== matlab function pmpc_mil_nu/减振器正模型（1000Hz）/MATLAB Function2 ==
  data: t input; F output; Temp_C input; cmpD input; cmpRD input; I_cmd input; cid input
function F = fwd_mf(t, Temp_C, cmpD, cmpRD, I_cmd, cid)
%#codegen
F = fwd_mf_impl(t, Temp_C, cmpD, cmpRD, I_cmd, cid);

== matlab function pmpc_mil_nu/减振器正模型（1000Hz）/MATLAB Function3 ==
  data: t input; F output; Temp_C input; cmpD input; cmpRD input; I_cmd input; cid input
function F = fwd_mf(t, Temp_C, cmpD, cmpRD, I_cmd, cid)
%#codegen
F = fwd_mf_impl(t, Temp_C, cmpD, cmpRD, I_cmd, cid);

== matlab function pmpc_mil_nu/减振器正模型（1000Hz）/MATLAB Function4 ==
  data: t input; F output; Temp_C input; cmpD input; cmpRD input; I_cmd input; cid input
function F = fwd_mf(t, Temp_C, cmpD, cmpRD, I_cmd, cid)
%#codegen
F = fwd_mf_impl(t, Temp_C, cmpD, cmpRD, I_cmd, cid);
